simulink model "nms_sim_2D_cost"  (R2024b)
settings: Solver=ode15s  StartTime=0.0  StopTime=t_sim  MaxStep=dt_max  EnableMultiTasking=on
values from neighbouring files (symbols this model uses):
  a_BFSH = param_ctrl(35)*1    [setCtrlPar_optim_CPGreflex2001_2D.m]
  a_GAS = param_ctrl(37)*1    [setCtrlPar_optim_CPGreflex2001_2D.m]
  a_GLU = param_ctrl(31)*1    [setCtrlPar_optim_CPGreflex2001_2D.m]
  a_HAM = param_ctrl(33)*1    [setCtrlPar_optim_CPGreflex2001_2D.m]
  a_HFL = param_ctrl(32)*1    [setCtrlPar_optim_CPGreflex2001_2D.m]
  a_RF = param_ctrl(34)*1    [setCtrlPar_optim_CPGreflex2001_2D.m]
  a_SOL = param_ctrl(38)*1    [setCtrlPar_optim_CPGreflex2001_2D.m]
  a_TA = param_ctrl(39)*1    [setCtrlPar_optim_CPGreflex2001_2D.m]
  a_VAS = param_ctrl(36)*1    [setCtrlPar_optim_CPGreflex2001_2D.m]
  ai = param_ctrl(96)*2.0    [setCtrlPar_optim_CPGreflex2001_2D.m]
  b_BFSH = param_ctrl(52)*.51    [setCtrlPar_optim_CPGreflex2001_2D.m]
  b_BFSHGAS = param_ctrl(55)*.51    [setCtrlPar_optim_CPGreflex2001_2D.m]
  b_BFSHHAM = param_ctrl(54)*.51    [setCtrlPar_optim_CPGreflex2001_2D.m]
  b_BFSHVAS = param_ctrl(53)*.51    [setCtrlPar_optim_CPGreflex2001_2D.m]
  b_GAS = param_ctrl(59)*.51    [setCtrlPar_optim_CPGreflex2001_2D.m]
  b_GASBFSH = param_ctrl(60)*.51    [setCtrlPar_optim_CPGreflex2001_2D.m]
  b_GASSOL = param_ctrl(61)*.51    [setCtrlPar_optim_CPGreflex2001_2D.m]
  b_GLU = param_ctrl(40)*.51    [setCtrlPar_optim_CPGreflex2001_2D.m]
  b_GLUHAM = param_ctrl(42)*.51    [setCtrlPar_optim_CPGreflex2001_2D.m]
  b_GLUHFL = param_ctrl(41)*.51    [setCtrlPar_optim_CPGreflex2001_2D.m]
  b_HAM = param_ctrl(46)*.51    [setCtrlPar_optim_CPGreflex2001_2D.m]
  b_HAMBFSH = param_ctrl(48)*.51    [setCtrlPar_optim_CPGreflex2001_2D.m]
  b_HAMGLU = param_ctrl(47)*.51    [setCtrlPar_optim_CPGreflex2001_2D.m]
  b_HFL = param_ctrl(43)*.51    [setCtrlPar_optim_CPGreflex2001_2D.m]
  b_HFLGLU = param_ctrl(44)*.51    [setCtrlPar_optim_CPGreflex2001_2D.m]
  b_HFLRF = param_ctrl(45)*.51    [setCtrlPar_optim_CPGreflex2001_2D.m]
  b_RF = param_ctrl(49)*.51    [setCtrlPar_optim_CPGreflex2001_2D.m]
  b_RFHFL = param_ctrl(50)*.51    [setCtrlPar_optim_CPGreflex2001_2D.m]
  b_RFVAS = param_ctrl(51)*.51    [setCtrlPar_optim_CPGreflex2001_2D.m]
  b_SOL = param_ctrl(62)*.51    [setCtrlPar_optim_CPGreflex2001_2D.m]
  b_SOLGAS = param_ctrl(64)*.51    [setCtrlPar_optim_CPGreflex2001_2D.m]
  b_SOLTA = param_ctrl(63)*.51    [setCtrlPar_optim_CPGreflex2001_2D.m]
  b_TA = param_ctrl(65)*.51    [setCtrlPar_optim_CPGreflex2001_2D.m]
  b_TASOL = param_ctrl(66)*.51    [setCtrlPar_optim_CPGreflex2001_2D.m]
  b_VAS = param_ctrl(56)*.51    [setCtrlPar_optim_CPGreflex2001_2D.m]
  b_VASBFSH = param_ctrl(57)*.51    [setCtrlPar_optim_CPGreflex2001_2D.m]
  b_VASRF = param_ctrl(58)*.51    [setCtrlPar_optim_CPGreflex2001_2D.m]
  bias = param_ctrl(97)*2.5    [setCtrlPar_optim_CPGreflex2001_2D.m]
  c = 0.05    [nms_MS_2D_scaled.m]
  c_jointstop = 0.3 / (pi/180)    (= 17.1887338539)    [nms_MS_2D_scaled.m]
  D12_F = 0.16    *scaleL_JPhys    [nms_MechInit_2D_scaleSkel.m]
  D12_S = 0.2460	*sub_height    [nms_MechInit_2D_scaleSkel.m]
  D12_T = 0.2450  *sub_height    [nms_MechInit_2D_scaleSkel.m]
  D12y_F = 0.039  *sub_height    [nms_MechInit_2D_scaleSkel.m]
  D12z_HAT = 0.1    [nms_MS_2D_scaled.m]
  D13_F = 0.20    *scaleL_JPhys    [nms_MechInit_2D_scaleSkel.m]
  D1G_F = 0.14    *scaleL_JPhys    [nms_MechInit_2D_scaleSkel.m]
  D1G_HAT = 0.35  *scaleL_JPhys    [nms_MechInit_2D_scaleSkel.m]
  D1G_S = (0.3 - D12y_F/4)	*scaleL_JPhys    [nms_MechInit_2D_scaleSkel.m]
  D1G_T = (0.3 - D12y_F/4)	*scaleL_JPhys    [nms_MechInit_2D_scaleSkel.m]
  D1Gy_F = D12y_F*D1G_F/D12_F    (= 0.07)    [nms_MechInit_2D_scaleSkel.m]
  d_BFSH = param_ctrl(26)*1    [setCtrlPar_optim_CPGreflex2001_2D.m]
  d_GAS = param_ctrl(28)*1    [setCtrlPar_optim_CPGreflex2001_2D.m]
  d_GLU = param_ctrl(22)*1    [setCtrlPar_optim_CPGreflex2001_2D.m]
  d_HAM = param_ctrl(24)*1    [setCtrlPar_optim_CPGreflex2001_2D.m]
  d_HFL = param_ctrl(23)*1    [setCtrlPar_optim_CPGreflex2001_2D.m]
  d_RF = param_ctrl(25)*1    [setCtrlPar_optim_CPGreflex2001_2D.m]
  d_SOL = param_ctrl(29)*1    [setCtrlPar_optim_CPGreflex2001_2D.m]
  d_TA = param_ctrl(30)*1    [setCtrlPar_optim_CPGreflex2001_2D.m]
  d_VAS = param_ctrl(27)*1    [setCtrlPar_optim_CPGreflex2001_2D.m]
  DeltaThRef = 5e-3    (= 0.005)    [nms_MS_2D_scaled.m]
  dloptBFSH = 3.0    (= 3)    [setCtrlPar_optim_CPGreflex2001_2D.m]
  dloptGAS = 3.0    (= 3)    [setCtrlPar_optim_CPGreflex2001_2D.m]
  dloptGLU = 3.0    (= 3)    [setCtrlPar_optim_CPGreflex2001_2D.m]
  dloptHAM = 3.0    (= 3)    [setCtrlPar_optim_CPGreflex2001_2D.m]
  dloptHFL = 3.0    (= 3)    [setCtrlPar_optim_CPGreflex2001_2D.m]
  dloptRF = 3.0    (= 3)    [setCtrlPar_optim_CPGreflex2001_2D.m]
  dloptSOL = 3.0    (= 3)    [setCtrlPar_optim_CPGreflex2001_2D.m]
  dloptTA = 3.0    (= 3)    [setCtrlPar_optim_CPGreflex2001_2D.m]
  dloptVAS = 3.0    (= 3)    [setCtrlPar_optim_CPGreflex2001_2D.m]
  ec_BFSH = param_ctrl(80)*0.15    [setCtrlPar_optim_CPGreflex2001_2D.m]
  ec_GAS = param_ctrl(82)*0.15    [setCtrlPar_optim_CPGreflex2001_2D.m]
  ec_GLU = param_ctrl(76)*0.15    [setCtrlPar_optim_CPGreflex2001_2D.m]
  ec_HAM = param_ctrl(78)*0.15    [setCtrlPar_optim_CPGreflex2001_2D.m]
  ec_HFL = param_ctrl(77)*0.15    [setCtrlPar_optim_CPGreflex2001_2D.m]
  ec_RF = param_ctrl(79)*0.15    [setCtrlPar_optim_CPGreflex2001_2D.m]
  ec_TA = param_ctrl(84)*0.15    [setCtrlPar_optim_CPGreflex2001_2D.m]
  ec_VAS = param_ctrl(81)*0.15    [setCtrlPar_optim_CPGreflex2001_2D.m]
  eref = 0.04    [nms_MS_2D_scaled.m]
  eref_GAS = 0.1    [nms_MS_2D_scaled.m]
  eref_SOL = 0.1    [nms_MS_2D_scaled.m]
  es_BFSH = param_ctrl(89)*0.15    [setCtrlPar_optim_CPGreflex2001_2D.m]
  es_GAS = param_ctrl(91)*0.15    [setCtrlPar_optim_CPGreflex2001_2D.m]
  es_GLU = param_ctrl(85)*0.15    [setCtrlPar_optim_CPGreflex2001_2D.m]
  es_HAM = param_ctrl(87)*0.15    [setCtrlPar_optim_CPGreflex2001_2D.m]
  es_HFL = param_ctrl(86)*0.15    [setCtrlPar_optim_CPGreflex2001_2D.m]
  es_RF = param_ctrl(88)*0.15    [setCtrlPar_optim_CPGreflex2001_2D.m]
  es_TA = param_ctrl(93)*0.15    [setCtrlPar_optim_CPGreflex2001_2D.m]
  es_VAS = param_ctrl(90)*0.15    [setCtrlPar_optim_CPGreflex2001_2D.m]
  FmaxBFSH = 350    [nms_MS_2D_scaled.m]
  FmaxGAS = 2000    [nms_MS_2D_scaled.m]
  FmaxGLU = 4000    [nms_MS_2D_scaled.m]
  FmaxHAM = 2000    [nms_MS_2D_scaled.m]
  FmaxHFL = 2000    [nms_MS_2D_scaled.m]
  FmaxRF = 850    [nms_MS_2D_scaled.m]
  FmaxSOL = 4000    [nms_MS_2D_scaled.m]
  FmaxTA = 800    [nms_MS_2D_scaled.m]
  FmaxVAS = 5000    [nms_MS_2D_scaled.m]
  g = 9.81    [nms_MS_2D_scaled.m]
  gamma_4 = param_ctrl(11) * 1.7    [setCtrlPar_optim_CPGreflexsynergy2023_2D.m]
  h_BFSH = param_ctrl(71)*.1    [setCtrlPar_optim_CPGreflex2001_2D.m]
  h_GAS = param_ctrl(73)*.1    [setCtrlPar_optim_CPGreflex2001_2D.m]
  h_GLU = param_ctrl(67)*.1    [setCtrlPar_optim_CPGreflex2001_2D.m]
  h_HAM = param_ctrl(69)*.1    [setCtrlPar_optim_CPGreflex2001_2D.m]
  h_HFL = param_ctrl(68)*.1    [setCtrlPar_optim_CPGreflex2001_2D.m]
  h_RF = param_ctrl(70)*.1    [setCtrlPar_optim_CPGreflex2001_2D.m]
  h_SOL = param_ctrl(74)*.1    [setCtrlPar_optim_CPGreflex2001_2D.m]
  h_TA = param_ctrl(75)*.1    [setCtrlPar_optim_CPGreflex2001_2D.m]
  h_VAS = param_ctrl(72)*.1    [setCtrlPar_optim_CPGreflex2001_2D.m]
  HLCtrlPar = [theta_tgt l_clr alpha_tgt alpha_cd alpha_cv]    [setCtrlPar_optim_reflex2015_2D.m]
  In_F = 0.005    *scaleM*scaleL_JPhys^2    [nms_MechInit_2D_scaleSkel.m]
  In_HAT = 2.5    *scaleM*scaleL_JPhys^2    [nms_MechInit_2D_scaleSkel.m]
  In_S = 0.05     *scaleM*scaleL_JPhys^2    [nms_MechInit_2D_scaleSkel.m]
  In_T = 0.15     *scaleM*scaleL_JPhys^2    [nms_MechInit_2D_scaleSkel.m]
  init_exc = 0.01    [setInitPar_optim_2D.m]
  init_fm = 0.01    [setInitPar_optim_2D.m]
  init_lce = 1    [setInitPar_optim_2D.m]
  init_LCPG = param_ctrl(12) * 0.01    [setCtrlPar_optim_CPGreflexsynergy2023_2D.m]
  init_LStance = 1    [setInitPar_optim_2D.m]
  init_N1 = osc_signal1(phi_off_osc_ind)    [setCtrlPar_optim_CPGreflex2001_2D.m]
  ... (+441 more)
undefined symbols (not defined in the file or in its folder): cost_act_exponent, cost_v_tgt, flag_controller, Newton, nStep_obj, nStep_startKin, Raphson, sgn, SSW_kin, terrain_slope_angle, v_plateS1, X, Y, Z
libraries: nesl_utility x94, sm_lib x90, simulink x28, simulink_extras x12
(part 12 of 20)

== system nms_sim_2D_cost/Muscle Actuation/R RF Link ==
  note: RF Attachment
  phi34 [rad] : Inport
  phi23 [rad] : Inport  Port=2
  Constant1 : Constant  Value=phimaxRFk
  Constant2 : Constant  Value=phirefRFk
  Constant3 : Constant  Value=rRFh
  Constant4 : Constant  Value=lslackRF+loptRF
  Constant5 : Constant  Value=phirefRFh
  Demux : Demux  Outputs=2
  Gain1 : Gain  Gain=rRFkmax
  Gain2 : Gain  Gain=rhoRFh
  Gain3 : Gain  Gain=phiScaleRFk
  Gain4 : Gain  Gain=rhoRFk/phiScaleRFk
  Gain5 : Gain  Gain=phiScaleRFk
  Mux : Mux  Inputs=2
  Product : Product  RndMeth=Zero
  Sum1 : Sum  Inputs=-+
  Sum2 : Sum  Inputs=|+-
  Sum3 : Sum  Inputs=-+|
  Sum4 : Sum  Inputs=|+-
  Sum5 : Sum  Inputs=++-
  length change term : Trigonometry
  offset correction term : Trigonometry
  variable lever term : Trigonometry  Operator=cos
  lmtu [m] : Outport  VectorParamsAs1DForOutWhenUnconnected=off
  lever34 [m] : Outport  Port=2  VectorParamsAs1DForOutWhenUnconnected=off
  lever23 [m] : Outport  Port=3  VectorParamsAs1DForOutWhenUnconnected=off
  wires:
  Sum5/1 -> lmtu [m]/1
  Constant4/1 -> Sum5/2
  Gain4/1 -> Sum5/3
  Gain2/1 -> Sum5/1
  phi34 [rad]/1 -> Sum4/1
  Constant5/1 -> Sum4/2
  Sum4/1 -> Product/1
  Constant3/1 -> Product/2, lever34 [m]/1
  Product/1 -> Gain2/1
  phi23 [rad]/1 -> Sum3/2
  Sum3/1 -> Gain3/1
  Constant1/1 -> Sum3/1, Sum2/2
  Sum2/1 -> Gain5/1
  Constant2/1 -> Sum2/1
  length change term/1 -> Sum1/2
  offset correction term/1 -> Sum1/1
  Sum1/1 -> Mux/1
  variable lever term/1 -> Mux/2
  Mux/1 -> Gain1/1
  Gain1/1 -> Demux/1
  Demux/2 -> lever23 [m]/1
  Demux/1 -> Gain4/1
  Gain3/1 -> variable lever term/1, length change term/1
  Gain5/1 -> offset correction term/1

== system nms_sim_2D_cost/Muscle Actuation/R SOL ==
  note: SOLEUS Muscle-Tendon Dynamics
  note: Excitation Contraction Coupling
  A : Inport
  lmtc [m] : Inport  Port=2
  eref : Inport  Port=3
  1 : Product  Inputs=**  InputSameDT=on  SaturateOnIntegerOverflow=on  OutDataTypeStr=Inherit: Same as first input
  1/lslack : Gain  Gain=1/lslackSOL  SaturateOnIntegerOverflow=on  OutDataTypeStr=Inherit: Same as input  ParamDataTypeStr=Inherit: Same as input
  BE force-length relation : Subsystem
  CE force-length relation : Subsystem
  CE inverse force-velocity relation : Subsystem
  Constant : Constant  Value=lslackSOL
  Fmax : Gain  Gain=FmaxSOL  SaturateOnIntegerOverflow=on  OutDataTypeStr=Inherit: Same as input  ParamDataTypeStr=Inherit: Same as input
  Fmax1 : Gain  Gain=FmaxSOL  SaturateOnIntegerOverflow=on  OutDataTypeStr=Inherit: Same as input  ParamDataTypeStr=Inherit: Same as input
  "Fpe = F^*pe * fv " : Product  InputSameDT=on  SaturateOnIntegerOverflow=on  OutDataTypeStr=Inherit: Same as first input
  Fv = Fse / (A*Fce) : Product  Inputs=*/  InputSameDT=on  SaturateOnIntegerOverflow=on  OutDataTypeStr=Inherit: Same as first input
  Integrator : Integrator  InitialConditionSource=external  LowerSaturationLimit=0.05
  PE force-length relation : Subsystem
  SE force-length relation : Subsystem
  Sum : Sum  Inputs=|+-  InputSameDT=on  SaturateOnIntegerOverflow=on  OutDataTypeStr=Inherit: Same as first input
  Sum1 : Sum  Inputs=|+-  InputSameDT=on  SaturateOnIntegerOverflow=on  OutDataTypeStr=Inherit: Same as first input
  Sum2 : Sum  Inputs=|-+  InputSameDT=on  SaturateOnIntegerOverflow=on  OutDataTypeStr=Inherit: Same as first input
  Sum3 : Sum  InputSameDT=on  SaturateOnIntegerOverflow=on  OutDataTypeStr=Inherit: Same as first input
  Sum4 : Sum  InputSameDT=on  SaturateOnIntegerOverflow=on  OutDataTypeStr=Inherit: Same as first input
  lce/lopt : Gain  Gain=1/loptSOL  SaturateOnIntegerOverflow=on  OutDataTypeStr=Inherit: Same as input  ParamDataTypeStr=Inherit: Same as input
  vmax*lopt : Gain  Gain=vmaxSOL*loptSOL  SaturateOnIntegerOverflow=on  OutDataTypeStr=Inherit: Same as input  ParamDataTypeStr=Inherit: Same as input
  Fmtc : Outport  InitialOutput=0  VectorParamsAs1DForOutWhenUnconnected=off
  Lce : Outport  Port=2  InitialOutput=0  VectorParamsAs1DForOutWhenUnconnected=off
  Vce : Outport  Port=3  InitialOutput=0  VectorParamsAs1DForOutWhenUnconnected=off
  Fce : Outport  Port=4  InitialOutput=0  VectorParamsAs1DForOutWhenUnconnected=off
  lse [m] : Outport  Port=5  InitialOutput=0  VectorParamsAs1DForOutWhenUnconnected=off
  wires:
  Integrator/1 -> Sum/2, lce/lopt/1, Lce/1  "lce"
  lce/lopt/1 -> CE force-length relation/1(lce [lopt]), PE force-length relation/1(lce [lopt]), BE force-length relation/1(lce [lopt])
  Fv = Fse / (A*Fce)/1 -> "Fpe = F^*pe * fv "/1, CE inverse force-velocity relation/1(Fv[Fmax])  "fv"
  vmax*lopt/1 -> Integrator/1, Vce/1  "vce"
  lmtc [m]/1 -> Sum2/2, Sum/1  "lmtc"
  Fmax/1 -> Fmtc/1  "Fmtc"
  1/lslack/1 -> SE force-length relation/1(lse [lslack])
  SE force-length relation/1(fse [Fmax]) -> Fmax/1, Sum4/1
  Sum2/1 -> Integrator/2
  Constant/1 -> Sum2/1
  CE force-length relation/1(fce [Fmax]) -> 1/1
  PE force-length relation/1(fpe [Fmax]) -> "Fpe = F^*pe * fv "/2, Sum3/1
  1/1 -> Sum3/2
  BE force-length relation/1(fbe [Fmax]) -> Sum4/2
  Sum3/1 -> Fv = Fse / (A*Fce)/2
  CE inverse force-velocity relation/1(v[vmax]) -> vmax*lopt/1
  A/1 -> 1/2
  Sum4/1 -> Sum1/1, Fv = Fse / (A*Fce)/1  "Fse+Fbe"
  "Fpe = F^*pe * fv "/1 -> Sum1/2
  Sum1/1 -> Fmax1/1  "Fse+Fbe-Fpe"
  Fmax1/1 -> Fce/1
  Sum/1 -> lse [m]/1, 1/lslack/1  "lse"
  eref/1 -> SE force-length relation/2(eref)

== system nms_sim_2D_cost/Muscle Actuation/R SOL Link ==
  note: Soleus Attachment
  phi12 [rad] : Inport
  Constant : Constant  Value=lslackSOL+loptSOL
  Constant3 : Constant  Value=phimaxSOL
  Constant5 : Constant  Value=phirefSOL
  Demux1 : Demux  Outputs=2
  Gain2 : Gain  Gain=rSOLmax
  Gain3 : Gain  Gain=phiScaleSOL
  Gain8 : Gain  Gain=phiScaleSOL
  Gain9 : Gain  Gain=rhoSOL/phiScaleSOL
  Mux1 : Mux  Inputs=2
  Sum4 : Sum  Inputs=-+
  Sum5 : Sum  Inputs=|+-
  Sum6 : Sum  Inputs=|+-
  Sum7 : Sum  Inputs=-+|
  length change term1 : Trigonometry
  offset correction term1 : Trigonometry
  variable lever term1 : Trigonometry  Operator=cos
  lmtc [m] : Outport  VectorParamsAs1DForOutWhenUnconnected=off
  lever [m] : Outport  Port=2  VectorParamsAs1DForOutWhenUnconnected=off
  wires:
  Constant/1 -> Sum5/1
  Sum5/1 -> lmtc [m]/1
  Gain9/1 -> Sum5/2
  Demux1/1 -> Gain9/1
  Demux1/2 -> lever [m]/1
  phi12 [rad]/1 -> Sum7/2
  Sum7/1 -> Gain3/1
  Constant3/1 -> Sum7/1, Sum6/2
  Sum6/1 -> Gain8/1
  Constant5/1 -> Sum6/1
  length change term1/1 -> Sum4/2
  offset correction term1/1 -> Sum4/1
  Sum4/1 -> Mux1/1
  variable lever term1/1 -> Mux1/2
  Mux1/1 -> Gain2/1
  Gain2/1 -> Demux1/1
  Gain3/1 -> variable lever term1/1, length change term1/1
  Gain8/1 -> offset correction term1/1

== system nms_sim_2D_cost/Muscle Actuation/R TA Link ==
  note: Muscle Length and Moment Arm
  phi12 [rad] : Inport
  Constant : Constant  Value=lslackTA+loptTA
  Constant3 : Constant  Value=phimaxTA
  Constant5 : Constant  Value=phirefTA
  Demux1 : Demux  Outputs=2
  Gain2 : Gain  Gain=rTAmax
  Gain3 : Gain  Gain=phiScaleTA
  Gain8 : Gain  Gain=phiScaleTA
  Gain9 : Gain  Gain=rhoTA/phiScaleTA
  Mux1 : Mux  Inputs=2
  Sum4 : Sum  Inputs=-+
  Sum5 : Sum  Inputs=|++
  Sum6 : Sum  Inputs=|+-
  Sum7 : Sum  Inputs=-+|
  length change term1 : Trigonometry
  offset correction term1 : Trigonometry
  variable lever term1 : Trigonometry  Operator=cos
  lmtc [m] : Outport  VectorParamsAs1DForOutWhenUnconnected=off
  lever [m] : Outport  Port=2  VectorParamsAs1DForOutWhenUnconnected=off
  wires:
  Constant/1 -> Sum5/1
  Sum5/1 -> lmtc [m]/1
  Gain9/1 -> Sum5/2
  Demux1/1 -> Gain9/1
  Demux1/2 -> lever [m]/1
  phi12 [rad]/1 -> Sum7/2
  Sum7/1 -> Gain3/1
  Constant3/1 -> Sum7/1, Sum6/2
  Sum6/1 -> Gain8/1
  Constant5/1 -> Sum6/1
  length change term1/1 -> Sum4/2
  offset correction term1/1 -> Sum4/1
  Sum4/1 -> Mux1/1
  variable lever term1/1 -> Mux1/2
  Mux1/1 -> Gain2/1
  Gain2/1 -> Demux1/1
  Gain3/1 -> variable lever term1/1, length change term1/1
  Gain8/1 -> offset correction term1/1

== system nms_sim_2D_cost/Muscle Actuation/R VAS Link ==
  note: Muscle Length and Moment Arm
  phi23 [rad] : Inport
  Constant : Constant  Value=lslackVAS+loptVAS
  Constant1 : Constant  Value=phimaxVAS
  Constant2 : Constant  Value=phirefVAS
  Demux : Demux  Outputs=2
  Gain1 : Gain  Gain=rVASmax
  Gain3 : Gain  Gain=phiScaleVAS
  Gain4 : Gain  Gain=rhoVAS/phiScaleVAS
  Gain5 : Gain  Gain=phiScaleVAS
  Mux : Mux  Inputs=2
  Sum1 : Sum  Inputs=-+
  Sum2 : Sum  Inputs=|+-
  Sum3 : Sum  Inputs=-+|
  Sum5 : Sum  Inputs=|+-
  length change term : Trigonometry
  offset correction term : Trigonometry
  variable lever term : Trigonometry  Operator=cos
  lmtu [m] : Outport  VectorParamsAs1DForOutWhenUnconnected=off
  lever [m] : Outport  Port=2  VectorParamsAs1DForOutWhenUnconnected=off
  wires:
  Constant/1 -> Sum5/1
  Sum5/1 -> lmtu [m]/1
  phi23 [rad]/1 -> Sum3/2
  Sum3/1 -> Gain3/1
  Constant1/1 -> Sum3/1, Sum2/2
  Sum2/1 -> Gain5/1
  Constant2/1 -> Sum2/1
  length change term/1 -> Sum1/2
  offset correction term/1 -> Sum1/1
  Sum1/1 -> Mux/1
  variable lever term/1 -> Mux/2
  Mux/1 -> Gain1/1
  Gain1/1 -> Demux/1
  Demux/2 -> lever [m]/1
  Demux/1 -> Gain4/1
  Gain3/1 -> variable lever term/1, length change term/1
  Gain5/1 -> offset correction term/1
  Gain4/1 -> Sum5/2

== system nms_sim_2D_cost/Muscle Actuation/RF ==
  note: Rectus Femoris Muscle-Tendon Dynamics
  note: Excitation Contraction Coupling
  A : Inport
  lmtc [m] : Inport  Port=2
  1 : Product  Inputs=**  InputSameDT=on  SaturateOnIntegerOverflow=on  OutDataTypeStr=Inherit: Same as first input
  1/lslack : Gain  Gain=1/lslackRF  SaturateOnIntegerOverflow=on  OutDataTypeStr=Inherit: Same as input  ParamDataTypeStr=Inherit: Same as input
  BE force-length relation : Subsystem
  CE force-length relation : Subsystem
  CE inverse force-velocity relation : Subsystem
  Constant : Constant  Value=lslackRF
  Fmax : Gain  Gain=FmaxRF  SaturateOnIntegerOverflow=on  OutDataTypeStr=Inherit: Same as input  ParamDataTypeStr=Inherit: Same as input
  Fmax1 : Gain  Gain=FmaxRF  SaturateOnIntegerOverflow=on  OutDataTypeStr=Inherit: Same as input  ParamDataTypeStr=Inherit: Same as input
  "Fpe = F^*pe * fv " : Product  InputSameDT=on  SaturateOnIntegerOverflow=on  OutDataTypeStr=Inherit: Same as first input
  Fv = Fse / (A*Fce) : Product  Inputs=*/  InputSameDT=on  SaturateOnIntegerOverflow=on  OutDataTypeStr=Inherit: Same as first input
  Integrator : Integrator  InitialConditionSource=external  LowerSaturationLimit=0.05
  PE force-length relation : Subsystem
  SE force-length relation : Subsystem
  Sum : Sum  Inputs=|+-  InputSameDT=on  SaturateOnIntegerOverflow=on  OutDataTypeStr=Inherit: Same as first input
  Sum1 : Sum  Inputs=|+-  InputSameDT=on  SaturateOnIntegerOverflow=on  OutDataTypeStr=Inherit: Same as first input
  Sum2 : Sum  Inputs=|-+  InputSameDT=on  SaturateOnIntegerOverflow=on  OutDataTypeStr=Inherit: Same as first input
  Sum3 : Sum  InputSameDT=on  SaturateOnIntegerOverflow=on  OutDataTypeStr=Inherit: Same as first input
  Sum4 : Sum  InputSameDT=on  SaturateOnIntegerOverflow=on  OutDataTypeStr=Inherit: Same as first input
  lce/lopt : Gain  Gain=1/loptRF  SaturateOnIntegerOverflow=on  OutDataTypeStr=Inherit: Same as input  ParamDataTypeStr=Inherit: Same as input
  vmax*lopt : Gain  Gain=vmaxRF*loptRF  SaturateOnIntegerOverflow=on  OutDataTypeStr=Inherit: Same as input  ParamDataTypeStr=Inherit: Same as input
  Fmtc : Outport  InitialOutput=0  VectorParamsAs1DForOutWhenUnconnected=off
  Lce : Outport  Port=2  InitialOutput=0  VectorParamsAs1DForOutWhenUnconnected=off
  Vce : Outport  Port=3  InitialOutput=0  VectorParamsAs1DForOutWhenUnconnected=off
  Fce : Outport  Port=4  InitialOutput=0  VectorParamsAs1DForOutWhenUnconnected=off
  lse [m] : Outport  Port=5  InitialOutput=0  VectorParamsAs1DForOutWhenUnconnected=off
  wires:
  Integrator/1 -> Sum/2, lce/lopt/1, Lce/1  "lce"
  lce/lopt/1 -> CE force-length relation/1(lce [lopt]), PE force-length relation/1(lce [lopt]), BE force-length relation/1(lce [lopt])
  Fv = Fse / (A*Fce)/1 -> "Fpe = F^*pe * fv "/1, CE inverse force-velocity relation/1(Fv[Fmax])  "fv"
  vmax*lopt/1 -> Integrator/1, Vce/1  "vce"
  lmtc [m]/1 -> Sum2/2, Sum/1  "lmtc"
  Fmax/1 -> Fmtc/1  "Fmtc"
  1/lslack/1 -> SE force-length relation/1(lse [lslack])
  SE force-length relation/1(fse [Fmax]) -> Fmax/1, Sum4/1
  Sum2/1 -> Integrator/2
  Constant/1 -> Sum2/1
  CE force-length relation/1(fce [Fmax]) -> 1/1
  PE force-length relation/1(fpe [Fmax]) -> Sum3/1, "Fpe = F^*pe * fv "/2
  1/1 -> Sum3/2
  BE force-length relation/1(fbe [Fmax]) -> Sum4/2
  Sum3/1 -> Fv = Fse / (A*Fce)/2
  CE inverse force-velocity relation/1(v[vmax]) -> vmax*lopt/1
  A/1 -> 1/2
  Sum4/1 -> Sum1/1, Fv = Fse / (A*Fce)/1  "Fse+Fbe"
  "Fpe = F^*pe * fv "/1 -> Sum1/2
  Sum1/1 -> Fmax1/1  "Fse+Fbe-Fpe"
  Fmax1/1 -> Fce/1
  Sum/1 -> lse [m]/1, 1/lslack/1  "lse"

== system nms_sim_2D_cost/Muscle Actuation/RF Link ==
  note: RF Attachment
  phi34 [rad] : Inport
  phi23 [rad] : Inport  Port=2
  Constant1 : Constant  Value=phimaxRFk
  Constant2 : Constant  Value=phirefRFk
  Constant3 : Constant  Value=rRFh
  Constant4 : Constant  Value=lslackRF+loptRF
  Constant5 : Constant  Value=phirefRFh
  Demux : Demux  Outputs=2
  Gain1 : Gain  Gain=rRFkmax
  Gain2 : Gain  Gain=rhoRFh
  Gain3 : Gain  Gain=phiScaleRFk
  Gain4 : Gain  Gain=rhoRFk/phiScaleRFk
  Gain5 : Gain  Gain=phiScaleRFk
  Mux : Mux  Inputs=2
  Product : Product  RndMeth=Zero
  Sum1 : Sum  Inputs=-+
  Sum2 : Sum  Inputs=|+-
  Sum3 : Sum  Inputs=-+|
  Sum4 : Sum  Inputs=|+-
  Sum5 : Sum  Inputs=++-
  length change term : Trigonometry
  offset correction term : Trigonometry
  variable lever term : Trigonometry  Operator=cos
  lmtu [m] : Outport  VectorParamsAs1DForOutWhenUnconnected=off
  lever34 [m] : Outport  Port=2  VectorParamsAs1DForOutWhenUnconnected=off
  lever23 [m] : Outport  Port=3  VectorParamsAs1DForOutWhenUnconnected=off
  wires:
  Sum5/1 -> lmtu [m]/1
  Constant4/1 -> Sum5/2
  Gain4/1 -> Sum5/3
  Gain2/1 -> Sum5/1
  phi34 [rad]/1 -> Sum4/1
  Constant5/1 -> Sum4/2
  Sum4/1 -> Product/1
  Constant3/1 -> Product/2, lever34 [m]/1
  Product/1 -> Gain2/1
  phi23 [rad]/1 -> Sum3/2
  Sum3/1 -> Gain3/1
  Constant1/1 -> Sum3/1, Sum2/2
  Sum2/1 -> Gain5/1
  Constant2/1 -> Sum2/1
  length change term/1 -> Sum1/2
  offset correction term/1 -> Sum1/1
  Sum1/1 -> Mux/1
  variable lever term/1 -> Mux/2
  Mux/1 -> Gain1/1
  Gain1/1 -> Demux/1
  Demux/2 -> lever23 [m]/1
  Demux/1 -> Gain4/1
  Gain3/1 -> variable lever term/1, length change term/1
  Gain5/1 -> offset correction term/1

== system nms_sim_2D_cost/Muscle Actuation/RF1 ==
  note: Rectus Femoris Muscle-Tendon Dynamics
  note: Excitation Contraction Coupling
  A : Inport
  lmtc [m] : Inport  Port=2
  1 : Product  Inputs=**  InputSameDT=on  SaturateOnIntegerOverflow=on  OutDataTypeStr=Inherit: Same as first input
  1/lslack : Gain  Gain=1/lslackRF  SaturateOnIntegerOverflow=on  OutDataTypeStr=Inherit: Same as input  ParamDataTypeStr=Inherit: Same as input
  BE force-length relation : Subsystem
  CE force-length relation : Subsystem
  CE inverse force-velocity relation : Subsystem
  Constant : Constant  Value=lslackRF
  Fmax : Gain  Gain=FmaxRF  SaturateOnIntegerOverflow=on  OutDataTypeStr=Inherit: Same as input  ParamDataTypeStr=Inherit: Same as input
  Fmax1 : Gain  Gain=FmaxRF  SaturateOnIntegerOverflow=on  OutDataTypeStr=Inherit: Same as input  ParamDataTypeStr=Inherit: Same as input
  "Fpe = F^*pe * fv " : Product  InputSameDT=on  SaturateOnIntegerOverflow=on  OutDataTypeStr=Inherit: Same as first input
  Fv = Fse / (A*Fce) : Product  Inputs=*/  InputSameDT=on  SaturateOnIntegerOverflow=on  OutDataTypeStr=Inherit: Same as first input
  Integrator : Integrator  InitialConditionSource=external  LowerSaturationLimit=0.05
  PE force-length relation : Subsystem
  SE force-length relation : Subsystem
  Sum : Sum  Inputs=|+-  InputSameDT=on  SaturateOnIntegerOverflow=on  OutDataTypeStr=Inherit: Same as first input
  Sum1 : Sum  Inputs=|+-  InputSameDT=on  SaturateOnIntegerOverflow=on  OutDataTypeStr=Inherit: Same as first input
  Sum2 : Sum  Inputs=|-+  InputSameDT=on  SaturateOnIntegerOverflow=on  OutDataTypeStr=Inherit: Same as first input
  Sum3 : Sum  InputSameDT=on  SaturateOnIntegerOverflow=on  OutDataTypeStr=Inherit: Same as first input
  Sum4 : Sum  InputSameDT=on  SaturateOnIntegerOverflow=on  OutDataTypeStr=Inherit: Same as first input
  lce/lopt : Gain  Gain=1/loptRF  SaturateOnIntegerOverflow=on  OutDataTypeStr=Inherit: Same as input  ParamDataTypeStr=Inherit: Same as input
  vmax*lopt : Gain  Gain=vmaxRF*loptRF  SaturateOnIntegerOverflow=on  OutDataTypeStr=Inherit: Same as input  ParamDataTypeStr=Inherit: Same as input
  Fmtc : Outport  InitialOutput=0  VectorParamsAs1DForOutWhenUnconnected=off
  Lce : Outport  Port=2  InitialOutput=0  VectorParamsAs1DForOutWhenUnconnected=off
  Vce : Outport  Port=3  InitialOutput=0  VectorParamsAs1DForOutWhenUnconnected=off
  Fce : Outport  Port=4  InitialOutput=0  VectorParamsAs1DForOutWhenUnconnected=off
  lse [m] : Outport  Port=5  InitialOutput=0  VectorParamsAs1DForOutWhenUnconnected=off
  wires:
  Integrator/1 -> Sum/2, lce/lopt/1, Lce/1  "lce"
  lce/lopt/1 -> CE force-length relation/1(lce [lopt]), PE force-length relation/1(lce [lopt]), BE force-length relation/1(lce [lopt])
  Fv = Fse / (A*Fce)/1 -> "Fpe = F^*pe * fv "/1, CE inverse force-velocity relation/1(Fv[Fmax])  "fv"
  vmax*lopt/1 -> Integrator/1, Vce/1  "vce"
  lmtc [m]/1 -> Sum2/2, Sum/1  "lmtc"
  Fmax/1 -> Fmtc/1  "Fmtc"
  1/lslack/1 -> SE force-length relation/1(lse [lslack])
  SE force-length relation/1(fse [Fmax]) -> Fmax/1, Sum4/1
  Sum2/1 -> Integrator/2
  Constant/1 -> Sum2/1
  CE force-length relation/1(fce [Fmax]) -> 1/1
  PE force-length relation/1(fpe [Fmax]) -> "Fpe = F^*pe * fv "/2, Sum3/1
  1/1 -> Sum3/2
  BE force-length relation/1(fbe [Fmax]) -> Sum4/2
  Sum3/1 -> Fv = Fse / (A*Fce)/2
  CE inverse force-velocity relation/1(v[vmax]) -> vmax*lopt/1
  A/1 -> 1/2
  Sum4/1 -> Sum1/1, Fv = Fse / (A*Fce)/1  "Fse+Fbe"
  "Fpe = F^*pe * fv "/1 -> Sum1/2
  Sum1/1 -> Fmax1/1  "Fse+Fbe-Fpe"
  Fmax1/1 -> Fce/1
  Sum/1 -> lse [m]/1, 1/lslack/1  "lse"

== system nms_sim_2D_cost/Muscle Actuation/TA1 ==
  note: Excitation Contraction Coupling
  note: SOLEUS Muscle-Tendon Dynamics
  A : Inport
  lmtc [m] : Inport  Port=2
  1 : Product  Inputs=**  InputSameDT=on  SaturateOnIntegerOverflow=on  OutDataTypeStr=Inherit: Same as first input
  1/lslack : Gain  Gain=1/lslackTA  SaturateOnIntegerOverflow=on  OutDataTypeStr=Inherit: Same as input  ParamDataTypeStr=Inherit: Same as input
  BE force-length relation : Subsystem
  CE force-length relation : Subsystem
  CE inverse force-velocity relation : Subsystem
  Constant : Constant  Value=lslackTA
  Fmax : Gain  Gain=FmaxTA  SaturateOnIntegerOverflow=on  OutDataTypeStr=Inherit: Same as input  ParamDataTypeStr=Inherit: Same as input
  Fmax1 : Gain  Gain=FmaxTA  SaturateOnIntegerOverflow=on  OutDataTypeStr=Inherit: Same as input  ParamDataTypeStr=Inherit: Same as input
  "Fpe = F^*pe * fv " : Product  InputSameDT=on  SaturateOnIntegerOverflow=on  OutDataTypeStr=Inherit: Same as first input
  Fv = Fse / (A*Fce) : Product  Inputs=*/  InputSameDT=on  SaturateOnIntegerOverflow=on  OutDataTypeStr=Inherit: Same as first input
  Integrator : Integrator  InitialConditionSource=external  LowerSaturationLimit=0.05
  PE force-length relation : Subsystem
  SE force-length relation : Subsystem
  Sum : Sum  Inputs=|+-  InputSameDT=on  SaturateOnIntegerOverflow=on  OutDataTypeStr=Inherit: Same as first input
  Sum1 : Sum  Inputs=|+-  InputSameDT=on  SaturateOnIntegerOverflow=on  OutDataTypeStr=Inherit: Same as first input
  Sum2 : Sum  Inputs=|-+  InputSameDT=on  SaturateOnIntegerOverflow=on  OutDataTypeStr=Inherit: Same as first input
  Sum3 : Sum  InputSameDT=on  SaturateOnIntegerOverflow=on  OutDataTypeStr=Inherit: Same as first input
  Sum4 : Sum  InputSameDT=on  SaturateOnIntegerOverflow=on  OutDataTypeStr=Inherit: Same as first input
  lce/lopt : Gain  Gain=1/loptTA  SaturateOnIntegerOverflow=on  OutDataTypeStr=Inherit: Same as input  ParamDataTypeStr=Inherit: Same as input
  vmax*lopt : Gain  Gain=vmaxTA*loptTA  SaturateOnIntegerOverflow=on  OutDataTypeStr=Inherit: Same as input  ParamDataTypeStr=Inherit: Same as input
  Fmtc : Outport  InitialOutput=0  VectorParamsAs1DForOutWhenUnconnected=off
  Lce : Outport  Port=2  InitialOutput=0  VectorParamsAs1DForOutWhenUnconnected=off
  Vce : Outport  Port=3  InitialOutput=0  VectorParamsAs1DForOutWhenUnconnected=off
  Fce : Outport  Port=4  InitialOutput=0  VectorParamsAs1DForOutWhenUnconnected=off
  lse [m] : Outport  Port=5  InitialOutput=0  VectorParamsAs1DForOutWhenUnconnected=off
  wires:
  CE inverse force-velocity relation/1(v[vmax]) -> vmax*lopt/1
  Sum3/1 -> Fv = Fse / (A*Fce)/2
  BE force-length relation/1(fbe [Fmax]) -> Sum4/2
  1/1 -> Sum3/2
  PE force-length relation/1(fpe [Fmax]) -> "Fpe = F^*pe * fv "/2, Sum3/1
  CE force-length relation/1(fce [Fmax]) -> 1/1
  Constant/1 -> Sum2/1
  Sum2/1 -> Integrator/2
  SE force-length relation/1(fse [Fmax]) -> Sum4/1, Fmax/1
  1/lslack/1 -> SE force-length relation/1(lse [lslack])
  Fmax/1 -> Fmtc/1  "Fmtc"
  lmtc [m]/1 -> Sum/1, Sum2/2  "lmtc"
  vmax*lopt/1 -> Integrator/1, Vce/1  "vce"
  Fv = Fse / (A*Fce)/1 -> "Fpe = F^*pe * fv "/1, CE inverse force-velocity relation/1(Fv[Fmax])  "fv"
  lce/lopt/1 -> PE force-length relation/1(lce [lopt]), BE force-length relation/1(lce [lopt]), CE force-length relation/1(lce [lopt])
  Integrator/1 -> lce/lopt/1, Sum/2, Lce/1  "lce"
  A/1 -> 1/2
  Sum4/1 -> Sum1/1, Fv = Fse / (A*Fce)/1  "Fse+Fbe"
  "Fpe = F^*pe * fv "/1 -> Sum1/2
  Sum1/1 -> Fmax1/1  "Fse+Fbe-Fpe"
  Fmax1/1 -> Fce/1
  Sum/1 -> lse [m]/1, 1/lslack/1  "lse"

== system nms_sim_2D_cost/Muscle Actuation/VAS ==
  note: VASTI Muscle-Tendon Dynamics
  note: Excitation Contraction Coupling
  A : Inport
  lmtc [m] : Inport  Port=2
  1 : Product  Inputs=**  InputSameDT=on  SaturateOnIntegerOverflow=on  OutDataTypeStr=Inherit: Same as first input
  1/lslack : Gain  Gain=1/lslackVAS  SaturateOnIntegerOverflow=on  OutDataTypeStr=Inherit: Same as input  ParamDataTypeStr=Inherit: Same as input
  BE force-length relation : Subsystem
  CE force-length relation : Subsystem
  CE inverse force-velocity relation : Subsystem
  Constant : Constant  Value=lslackVAS
  Fmax : Gain  Gain=FmaxVAS  SaturateOnIntegerOverflow=on  OutDataTypeStr=Inherit: Same as input  ParamDataTypeStr=Inherit: Same as input
  Fmax1 : Gain  Gain=FmaxVAS  SaturateOnIntegerOverflow=on  OutDataTypeStr=Inherit: Same as input  ParamDataTypeStr=Inherit: Same as input
  "Fpe = F^*pe * fv " : Product  InputSameDT=on  SaturateOnIntegerOverflow=on  OutDataTypeStr=Inherit: Same as first input
  Fv = Fse / (A*Fce) : Product  Inputs=*/  InputSameDT=on  SaturateOnIntegerOverflow=on  OutDataTypeStr=Inherit: Same as first input
  Integrator : Integrator  InitialConditionSource=external  LowerSaturationLimit=0.05
  PE force-length relation : Subsystem
  SE force-length relation : Subsystem
  Sum : Sum  Inputs=|+-  InputSameDT=on  SaturateOnIntegerOverflow=on  OutDataTypeStr=Inherit: Same as first input
  Sum1 : Sum  Inputs=|+-  InputSameDT=on  SaturateOnIntegerOverflow=on  OutDataTypeStr=Inherit: Same as first input
  Sum2 : Sum  Inputs=|-+  InputSameDT=on  SaturateOnIntegerOverflow=on  OutDataTypeStr=Inherit: Same as first input
  Sum3 : Sum  InputSameDT=on  SaturateOnIntegerOverflow=on  OutDataTypeStr=Inherit: Same as first input
  Sum4 : Sum  InputSameDT=on  SaturateOnIntegerOverflow=on  OutDataTypeStr=Inherit: Same as first input
  lce/lopt : Gain  Gain=1/loptVAS  SaturateOnIntegerOverflow=on  OutDataTypeStr=Inherit: Same as input  ParamDataTypeStr=Inherit: Same as input
  vmax*lopt : Gain  Gain=vmaxVAS*loptVAS  SaturateOnIntegerOverflow=on  OutDataTypeStr=Inherit: Same as input  ParamDataTypeStr=Inherit: Same as input
  Fmtc : Outport  InitialOutput=0  VectorParamsAs1DForOutWhenUnconnected=off
  Lce : Outport  Port=2  InitialOutput=0  VectorParamsAs1DForOutWhenUnconnected=off
  Vce : Outport  Port=3  InitialOutput=0  VectorParamsAs1DForOutWhenUnconnected=off
  Fce : Outport  Port=4  InitialOutput=0  VectorParamsAs1DForOutWhenUnconnected=off
  lse [m] : Outport  Port=5  InitialOutput=0  VectorParamsAs1DForOutWhenUnconnected=off
  wires:
  Integrator/1 -> Sum/2, lce/lopt/1, Lce/1  "lce"
  lce/lopt/1 -> CE force-length relation/1(lce [lopt]), PE force-length relation/1(lce [lopt]), BE force-length relation/1(lce [lopt])
  Fv = Fse / (A*Fce)/1 -> "Fpe = F^*pe * fv "/1, CE inverse force-velocity relation/1(Fv[Fmax])  "fv"
  vmax*lopt/1 -> Integrator/1, Vce/1  "vce"
  lmtc [m]/1 -> Sum2/2, Sum/1  "lmtc"
  Fmax/1 -> Fmtc/1  "Fmtc"
  1/lslack/1 -> SE force-length relation/1(lse [lslack])
  SE force-length relation/1(fse [Fmax]) -> Fmax/1, Sum4/1
  Sum2/1 -> Integrator/2
  Constant/1 -> Sum2/1
  CE force-length relation/1(fce [Fmax]) -> 1/1
  PE force-length relation/1(fpe [Fmax]) -> Sum3/1, "Fpe = F^*pe * fv "/2
  1/1 -> Sum3/2
  BE force-length relation/1(fbe [Fmax]) -> Sum4/2
  Sum3/1 -> Fv = Fse / (A*Fce)/2
  CE inverse force-velocity relation/1(v[vmax]) -> vmax*lopt/1
  A/1 -> 1/2
  Sum4/1 -> Sum1/1, Fv = Fse / (A*Fce)/1  "Fse+Fbe"
  "Fpe = F^*pe * fv "/1 -> Sum1/2
  Sum1/1 -> Fmax1/1  "Fse+Fbe-Fpe"
  Fmax1/1 -> Fce/1
  Sum/1 -> lse [m]/1, 1/lslack/1  "lse"

== system nms_sim_2D_cost/Muscle Actuation/VAS Link ==
  note: Muscle Length and Moment Arm
  phi23 [rad] : Inport
  Constant : Constant  Value=lslackVAS+loptVAS
  Constant1 : Constant  Value=phimaxVAS
  Constant2 : Constant  Value=phirefVAS
  Demux : Demux  Outputs=2
  Gain1 : Gain  Gain=rVASmax
  Gain3 : Gain  Gain=phiScaleVAS
  Gain4 : Gain  Gain=rhoVAS/phiScaleVAS
  Gain5 : Gain  Gain=phiScaleVAS
  Mux : Mux  Inputs=2
  Sum1 : Sum  Inputs=-+
  Sum2 : Sum  Inputs=|+-
  Sum3 : Sum  Inputs=-+|
  Sum5 : Sum  Inputs=|+-
  length change term : Trigonometry
  offset correction term : Trigonometry
  variable lever term : Trigonometry  Operator=cos
  lmtu [m] : Outport  VectorParamsAs1DForOutWhenUnconnected=off
  lever [m] : Outport  Port=2  VectorParamsAs1DForOutWhenUnconnected=off
  wires:
  Constant/1 -> Sum5/1
  Sum5/1 -> lmtu [m]/1
  phi23 [rad]/1 -> Sum3/2
  Sum3/1 -> Gain3/1
  Constant1/1 -> Sum3/1, Sum2/2
  Sum2/1 -> Gain5/1
  Constant2/1 -> Sum2/1
  length change term/1 -> Sum1/2
  offset correction term/1 -> Sum1/1
  Sum1/1 -> Mux/1
  variable lever term/1 -> Mux/2
  Mux/1 -> Gain1/1
  Gain1/1 -> Demux/1
  Demux/2 -> lever [m]/1
  Demux/1 -> Gain4/1
  Gain3/1 -> variable lever term/1, length change term/1
  Gain5/1 -> offset correction term/1
  Gain4/1 -> Sum5/2

== system nms_sim_2D_cost/Muscle Actuation/VAS1 ==
  note: VASTI Muscle-Tendon Dynamics
  note: Excitation Contraction Coupling
  A : Inport
  lmtc [m] : Inport  Port=2
  1 : Product  Inputs=**  InputSameDT=on  SaturateOnIntegerOverflow=on  OutDataTypeStr=Inherit: Same as first input
  1/lslack : Gain  Gain=1/lslackVAS  SaturateOnIntegerOverflow=on  OutDataTypeStr=Inherit: Same as input  ParamDataTypeStr=Inherit: Same as input
  BE force-length relation : Subsystem
  CE force-length relation : Subsystem
  CE inverse force-velocity relation : Subsystem
  Constant : Constant  Value=lslackVAS
  Fmax : Gain  Gain=FmaxVAS  SaturateOnIntegerOverflow=on  OutDataTypeStr=Inherit: Same as input  ParamDataTypeStr=Inherit: Same as input
  Fmax1 : Gain  Gain=FmaxVAS  SaturateOnIntegerOverflow=on  OutDataTypeStr=Inherit: Same as input  ParamDataTypeStr=Inherit: Same as input
  "Fpe = F^*pe * fv " : Product  InputSameDT=on  SaturateOnIntegerOverflow=on  OutDataTypeStr=Inherit: Same as first input
  Fv = Fse / (A*Fce) : Product  Inputs=*/  InputSameDT=on  SaturateOnIntegerOverflow=on  OutDataTypeStr=Inherit: Same as first input
  Integrator : Integrator  InitialConditionSource=external  LowerSaturationLimit=0.05
  PE force-length relation : Subsystem
  SE force-length relation : Subsystem
  Sum : Sum  Inputs=|+-  InputSameDT=on  SaturateOnIntegerOverflow=on  OutDataTypeStr=Inherit: Same as first input
  Sum1 : Sum  Inputs=|+-  InputSameDT=on  SaturateOnIntegerOverflow=on  OutDataTypeStr=Inherit: Same as first input
  Sum2 : Sum  Inputs=|-+  InputSameDT=on  SaturateOnIntegerOverflow=on  OutDataTypeStr=Inherit: Same as first input
  Sum3 : Sum  InputSameDT=on  SaturateOnIntegerOverflow=on  OutDataTypeStr=Inherit: Same as first input
  Sum4 : Sum  InputSameDT=on  SaturateOnIntegerOverflow=on  OutDataTypeStr=Inherit: Same as first input
  lce/lopt : Gain  Gain=1/loptVAS  SaturateOnIntegerOverflow=on  OutDataTypeStr=Inherit: Same as input  ParamDataTypeStr=Inherit: Same as input
  vmax*lopt : Gain  Gain=vmaxVAS*loptVAS  SaturateOnIntegerOverflow=on  OutDataTypeStr=Inherit: Same as input  ParamDataTypeStr=Inherit: Same as input
  Fmtc : Outport  InitialOutput=0  VectorParamsAs1DForOutWhenUnconnected=off
  Lce : Outport  Port=2  InitialOutput=0  VectorParamsAs1DForOutWhenUnconnected=off
  Vce : Outport  Port=3  InitialOutput=0  VectorParamsAs1DForOutWhenUnconnected=off
  Fce : Outport  Port=4  InitialOutput=0  VectorParamsAs1DForOutWhenUnconnected=off
  lse [m] : Outport  Port=5  InitialOutput=0  VectorParamsAs1DForOutWhenUnconnected=off
  wires:
  Integrator/1 -> Sum/2, lce/lopt/1, Lce/1  "lce"
  lce/lopt/1 -> CE force-length relation/1(lce [lopt]), PE force-length relation/1(lce [lopt]), BE force-length relation/1(lce [lopt])
  Fv = Fse / (A*Fce)/1 -> "Fpe = F^*pe * fv "/1, CE inverse force-velocity relation/1(Fv[Fmax])  "fv"
  vmax*lopt/1 -> Integrator/1, Vce/1  "vce"
  lmtc [m]/1 -> Sum2/2, Sum/1  "lmtc"
  Fmax/1 -> Fmtc/1  "Fmtc"
  1/lslack/1 -> SE force-length relation/1(lse [lslack])
  SE force-length relation/1(fse [Fmax]) -> Fmax/1, Sum4/1
  Sum2/1 -> Integrator/2
  Constant/1 -> Sum2/1
  CE force-length relation/1(fce [Fmax]) -> 1/1
  PE force-length relation/1(fpe [Fmax]) -> "Fpe = F^*pe * fv "/2, Sum3/1
  1/1 -> Sum3/2
  BE force-length relation/1(fbe [Fmax]) -> Sum4/2
  Sum3/1 -> Fv = Fse / (A*Fce)/2
  CE inverse force-velocity relation/1(v[vmax]) -> vmax*lopt/1
  A/1 -> 1/2
  Sum4/1 -> Sum1/1, Fv = Fse / (A*Fce)/1  "Fse+Fbe"
  "Fpe = F^*pe * fv "/1 -> Sum1/2
  Sum1/1 -> Fmax1/1  "Fse+Fbe-Fpe"
  Fmax1/1 -> Fce/1
  Sum/1 -> lse [m]/1, 1/lslack/1  "lse"

== system nms_sim_2D_cost/Muscle synergy Controller/Left Movement Generator ==
  note: Movement Generator
  P1 : Inport
  P2 : Inport  Port=2
  P3 : Inport  Port=3
  P4 : Inport  Port=4
  P5 : Inport  Port=5
  Demux : Demux  Outputs=3
  Demux1 : Demux  Outputs=2
  Demux2 : Demux  Outputs=5
  Demux3 : Demux  Outputs=2
  Demux4 : Demux
  Gain : Gain  Gain=w_GLU1
  Gain1 : Gain  Gain=w_VAS1
  Gain10 : Gain  Gain=w_TA4
  Gain11 : Gain  Gain=w_GLU5
  Gain12 : Gain  Gain=w_BFSH5
  Gain13 : Gain  Gain=w_RF5
  Gain14 : Gain  Gain=w_HFL3
  Gain15 : Gain  Gain=w_HAM5
  Gain2 : Gain  Gain=w_TA1
  Gain21 : Gain  Gain=pulseW1
  Gain22 : Gain  Gain=pulseW2
  Gain23 : Gain  Gain=pulseW3
  Gain24 : Gain  Gain=pulseW4
  Gain25 : Gain  Gain=pulseW5
  Gain3 : Gain  Gain=w_SOL2
  Gain4 : Gain  Gain=w_GAS2
  Gain5 : Gain  Gain=w_BFSH3
  Gain6 : Gain  Gain=w_TA3
  Gain7 : Gain  Gain=w_RF3
  Gain8 : Gain  Gain=w_GAS3
  Gain9 : Gain  Gain=w_VAS4
  Mux : Mux  Inputs=3
  Mux1 : Mux  Inputs=2
  Mux2 : Mux  Inputs=5
  Mux3 : Mux  Inputs=2
  Mux4 : Mux
  Sum{,1..2,5..6} (5 alike) : Sum
  Sum4 : Sum  Inputs=+++
  HFL : Outport
  GLU : Outport  Port=2
  HAM : Outport  Port=3
  VAS : Outport  Port=4
  RF : Outport  Port=5
  BFSH : Outport  Port=6
  GAS : Outport  Port=7
  SOL : Outport  Port=8
  TA : Outport  Port=9
  wires:
  Demux4/1 -> Sum/2  "GLU5"
  Sum6/1 -> RF/1
  Gain9/1 -> Mux3/1
  Demux2/1 -> HFL/1  "HF3"
  [Pulse3] -> Gain8/1, Gain7/1, Gain6/1, Gain5/1, Gain14/1
  [Pulse5] -> Gain15/1, Gain13/1, Gain12/1, Gain11/1
  Sum2/1 -> GAS/1
  Sum4/1 -> TA/1
  Demux2/3 -> Sum4/2  "TA3"
  Gain14/1 -> Mux2/1
  [P3_PulseAct] -> Demux2/1
  Gain7/1 -> Mux2/4
  Sum1/1 -> BFSH/1
  [Pulse4] -> Gain10/1, Gain9/1
  Mux2/1 -> [P3_PulseAct]
  Demux/3 -> Sum4/1  "TA1"
  Gain4/1 -> Mux1/2
  Sum/1 -> GLU/1
  Mux1/1 -> [P2_PulseAct]
  Gain13/1 -> Mux4/3
  [P4_PulseAct] -> Demux3/1
  Demux3/2 -> Sum4/3  "TA4"
  [P1_PulseAct] -> Demux/1
  Demux4/3 -> Sum6/2  "RF5"
  Demux4/4 -> HAM/1  "HAM5"
  Demux1/1 -> SOL/1  "SOL2"
  [Pulse2] -> Gain4/1, Gain3/1
  Sum5/1 -> VAS/1
  Gain11/1 -> Mux4/1
  Gain10/1 -> Mux3/2
  Gain1/1 -> Mux/2
  [P5_PulseAct] -> Demux4/1
  Demux4/2 -> Sum1/2  "BFSH5"
  Demux2/4 -> Sum6/1  "RF3"
  Gain3/1 -> Mux1/1
  Gain12/1 -> Mux4/2
  Gain5/1 -> Mux2/2
  Demux2/5 -> Sum2/2  "GAS3"
  Gain2/1 -> Mux/3
  Mux3/1 -> [P4_PulseAct]
  Gain6/1 -> Mux2/3
  Demux/2 -> Sum5/1  "VAS1"
  Gain8/1 -> Mux2/5
  Demux1/2 -> Sum2/1  "GAS2"
  [Pulse1] -> Gain2/1, Gain1/1, Gain/1
  Demux/1 -> Sum/1  "GLU1"
  Demux2/2 -> Sum1/1  "BFSH3"
  Mux4/1 -> [P5_PulseAct]
  Gain15/1 -> Mux4/4
  Mux/1 -> [P1_PulseAct]
  Gain/1 -> Mux/1
  Demux3/1 -> Sum5/2  "VAS4"
  [P2_PulseAct] -> Demux1/1
  Gain21/1 -> [Pulse1]
  Gain22/1 -> [Pulse2]
  Gain25/1 -> [Pulse5]
  Gain24/1 -> [Pulse4]
  Gain23/1 -> [Pulse3]
  P1/1 -> Gain21/1
  P2/1 -> Gain22/1
  P3/1 -> Gain23/1
  P4/1 -> Gain24/1
  P5/1 -> Gain25/1

== system nms_sim_2D_cost/Muscle synergy Controller/Left Movement Regulator ==
  note: Trunk Balance
  note: Speed Regulator
  theta : Inport
  dtheta : Inport  Port=2
  v : Inport  Port=3
  Stance : Inport  Port=4
  Left Speed Regulator : Subsystem
  Left Trunk Balance : Subsystem
  Product{,1..3} (4 alike) : Product
  LExcHFL_MR : Outport
  LExcGLU_MR : Outport  Port=2
  LExcTA_MR : Outport  Port=3
  LExcSOL_MR : Outport  Port=4
  wires:
  Stance/1 -> Product3/2, Product2/2, Left Speed Regulator/Enable, Product1/2, Product/2, Left Trunk Balance/Enable
  Left Trunk Balance/1(LExcHFL_MR) -> Product/1
  Left Trunk Balance/2(LExcGLU_MR) -> Product1/1
  Left Speed Regulator/1(LExcTA_MR) -> Product2/1
  Left Speed Regulator/2(LExcSOL_MR) -> Product3/1
  theta/1 -> Left Trunk Balance/1(theta)
  dtheta/1 -> Left Trunk Balance/2(dtheta)
  v/1 -> Left Speed Regulator/1(v)
  Product/1 -> LExcHFL_MR/1
  Product1/1 -> LExcGLU_MR/1
  Product2/1 -> LExcTA_MR/1
  Product3/1 -> LExcSOL_MR/1

== system nms_sim_2D_cost/Muscle synergy Controller/Right Movement Generator ==
  note: Movement Generator
  P1 : Inport
  P2 : Inport  Port=2
  P3 : Inport  Port=3
  P4 : Inport  Port=4
  P5 : Inport  Port=5
  Demux : Demux  Outputs=3
  Demux1 : Demux  Outputs=2
  Demux2 : Demux  Outputs=5
  Demux3 : Demux  Outputs=2
  Demux4 : Demux
  Gain : Gain  Gain=w_GLU1
  Gain1 : Gain  Gain=w_VAS1
  Gain10 : Gain  Gain=w_TA4
  Gain11 : Gain  Gain=w_GLU5
  Gain12 : Gain  Gain=w_BFSH5
  Gain13 : Gain  Gain=w_RF5
  Gain14 : Gain  Gain=w_HFL3
  Gain15 : Gain  Gain=w_HAM5
  Gain2 : Gain  Gain=w_TA1
  Gain21 : Gain  Gain=pulseW1
  Gain22 : Gain  Gain=pulseW2
  Gain23 : Gain  Gain=pulseW3
  Gain24 : Gain  Gain=pulseW4
  Gain25 : Gain  Gain=pulseW5
  Gain3 : Gain  Gain=w_SOL2
  Gain4 : Gain  Gain=w_GAS2
  Gain5 : Gain  Gain=w_BFSH3
  Gain6 : Gain  Gain=w_TA3
  Gain7 : Gain  Gain=w_RF3
  Gain8 : Gain  Gain=w_GAS3
  Gain9 : Gain  Gain=w_VAS4
  Mux : Mux  Inputs=3
  Mux1 : Mux  Inputs=2
  Mux2 : Mux  Inputs=5
  Mux3 : Mux  Inputs=2
  Mux4 : Mux
  Sum{,1..2,5..6} (5 alike) : Sum
  Sum4 : Sum  Inputs=+++
  HFL : Outport
  GLU : Outport  Port=2
  HAM : Outport  Port=3
  VAS : Outport  Port=4
  RF : Outport  Port=5
  BFSH : Outport  Port=6
  GAS : Outport  Port=7
  SOL : Outport  Port=8
  TA : Outport  Port=9
  wires:
  Demux4/1 -> Sum/2  "GLU5"
  Sum6/1 -> RF/1
  Gain9/1 -> Mux3/1
  Demux2/1 -> HFL/1  "HF3"
  [Pulse3] -> Gain8/1, Gain7/1, Gain6/1, Gain5/1, Gain14/1
  [Pulse5] -> Gain15/1, Gain13/1, Gain12/1, Gain11/1
  Sum2/1 -> GAS/1
  Sum4/1 -> TA/1
  Demux2/3 -> Sum4/2  "TA3"
  Gain14/1 -> Mux2/1
  [P3_PulseAct] -> Demux2/1
  Gain7/1 -> Mux2/4
  Sum1/1 -> BFSH/1
  [Pulse4] -> Gain10/1, Gain9/1
  Mux2/1 -> [P3_PulseAct]
  Demux/3 -> Sum4/1  "TA1"
  Gain4/1 -> Mux1/2
  Sum/1 -> GLU/1
  Mux1/1 -> [P2_PulseAct]
  Gain13/1 -> Mux4/3
  [P4_PulseAct] -> Demux3/1
  Demux3/2 -> Sum4/3  "TA4"
  [P1_PulseAct] -> Demux/1
  Demux4/3 -> Sum6/2  "RF5"
  Demux4/4 -> HAM/1  "HAM5"
  Demux1/1 -> SOL/1  "SOL2"
  [Pulse2] -> Gain4/1, Gain3/1
  Sum5/1 -> VAS/1
  Gain11/1 -> Mux4/1
  Gain10/1 -> Mux3/2
  Gain1/1 -> Mux/2
  [P5_PulseAct] -> Demux4/1
  Demux4/2 -> Sum1/2  "BFSH5"
  Demux2/4 -> Sum6/1  "RF3"
  Gain3/1 -> Mux1/1
  Gain12/1 -> Mux4/2
  Gain5/1 -> Mux2/2
  Demux2/5 -> Sum2/2  "GAS3"
  Gain2/1 -> Mux/3
  Mux3/1 -> [P4_PulseAct]
  Gain6/1 -> Mux2/3
  Demux/2 -> Sum5/1  "VAS1"
  Gain8/1 -> Mux2/5
  Demux1/2 -> Sum2/1  "GAS2"
  [Pulse1] -> Gain2/1, Gain1/1, Gain/1
  Demux/1 -> Sum/1  "GLU1"
  Demux2/2 -> Sum1/1  "BFSH3"
  Mux4/1 -> [P5_PulseAct]
  Gain15/1 -> Mux4/4
  Mux/1 -> [P1_PulseAct]
  Gain/1 -> Mux/1
  Demux3/1 -> Sum5/2  "VAS4"
  [P2_PulseAct] -> Demux1/1
  Gain21/1 -> [Pulse1]
  Gain22/1 -> [Pulse2]
  Gain25/1 -> [Pulse5]
  Gain24/1 -> [Pulse4]
  Gain23/1 -> [Pulse3]
  P1/1 -> Gain21/1
  P2/1 -> Gain22/1
  P3/1 -> Gain23/1
  P4/1 -> Gain24/1
  P5/1 -> Gain25/1

== system nms_sim_2D_cost/Muscle synergy Controller/Right Movement Regulator ==
  note: Speed Regulator
  note: Trunk Balance
  theta : Inport
  dtheta : Inport  Port=2
  v : Inport  Port=3
  Stance : Inport  Port=4
  Product{,1..3} (4 alike) : Product
  Right Speed Regulator : Subsystem
  Right Trunk Balance : Subsystem
  RExcHFL_MR : Outport
  RExcGLU_MR : Outport  Port=2
  RExcTA_MR : Outport  Port=3
  RExcSOL_MR : Outport  Port=4
  wires:
  Product3/1 -> RExcSOL_MR/1
  Product2/1 -> RExcTA_MR/1
  Product1/1 -> RExcGLU_MR/1
  Product/1 -> RExcHFL_MR/1
  v/1 -> Right Speed Regulator/1(v)
  dtheta/1 -> Right Trunk Balance/2(dtheta)
  theta/1 -> Right Trunk Balance/1(theta)
  Right Speed Regulator/2(RExcSOL_MR) -> Product3/1
  Right Speed Regulator/1(RExcTA_MR) -> Product2/1
  Right Trunk Balance/2(RExcGLU_MR) -> Product1/1
  Right Trunk Balance/1(RExcHFL_MR) -> Product/1
  Stance/1 -> Right Trunk Balance/Enable, Product/2, Product1/2, Right Speed Regulator/Enable, Product2/2, Product3/2

== system nms_sim_2D_cost/Reflex Controller/Higher Control Layer (Supraspinal Control) ==
  note: Higher Control Layer
      | (Supra Spinal Control)
  note: Stance to Swing Leg Decision
  note: Target Foot Placement
  note: Target Swing Leg Length
      | (constant)
  note: Target Trunk Angle
      | (constant)
  LL Delay{1..4} (4 alike) : TransportDelay  DelayTime=LongLoopDelay
  Mux1 : Mux  Inputs=3
  Mux6 : Mux  Inputs=3
  Selector{1..4} (4 alike) : Selector  InputPortWidth=3  IndexOptions=Index vector (dialog)  Indices=1  OutputSizes=1
  Stance to Swing : Subsystem
  Sum{1..2,7..8} (4 alike) : Sum  Inputs=-+|
  Terminator1 : Terminator
  alpha_tgt : Fcn  Expr=u(1) + u(2)*u(4) + u(3)*u(5)
  alpha_tgt1 : Fcn  Expr=u(1) + u(2)*u(4) + u(3)*u(5)
  tag scope: LSwInit=global, Lalpha_tgt=global, RSwInit=global, Ralpha_tgt=global, leg_clr=global, theta_tgt=global
  wires:
  LL Delay2/1 -> [RSwInit]
  LL Delay1/1 -> [LSwInit]
  [dd_theta] -> Sum7/1, Sum8/1
  [dd_Rphi23] -> Stance to Swing/8(Rphi23)
  [dd_Lphi23] -> Stance to Swing/5(Lphi23)
  [dd_Lphi34] -> Stance to Swing/4(Lphi34)
  Sum7/1 -> Stance to Swing/3(Lalpha_tgt)
  [dd_LStance] -> Stance to Swing/1(LStance)
  Sum8/1 -> Stance to Swing/6(Ralpha_tgt)
  Stance to Swing/1(LSwInit) -> LL Delay1/1
  [dd_RStance] -> Stance to Swing/2(RStance)
  Stance to Swing/3(RSwInit) -> LL Delay2/1
  [Ralpha_tgt] -> Sum8/2
  [Lalpha_tgt] -> Sum7/2
  Stance to Swing/2(Flight) -> Terminator1/1
  [dd_Rphi34] -> Stance to Swing/7(Rphi34)
  [leg_clr0] -> [leg_clr]
  [theta0] -> [theta_tgt]
  Sum1/1 -> Mux1/2  "d"
  LL Delay3/1 -> [Lalpha_tgt]
  Selector3/1 -> Mux6/3, Mux1/3
  alpha_tgt1/1 -> LL Delay4/1
  [alpha_par] -> Mux6/1, Mux1/1  "1~3"
  LL Delay4/1 -> [Ralpha_tgt]
  [dd_dxyzHAT] -> Selector3/1  "v"
  Mux1/1 -> alpha_tgt1/1
  Selector1/1 -> Sum2/2, Sum1/2
  [dd_xyzLShank1] -> Selector4/1
  Selector4/1 -> Sum1/1
  Mux6/1 -> alpha_tgt/1
  alpha_tgt/1 -> LL Delay3/1
  [dd_xyzRShank1] -> Selector2/1
  Sum2/1 -> Mux6/2  "d"
  [dd_xyzHAT] -> Selector1/1
  Selector2/1 -> Sum2/1
